simulink model "Main20210122"  (R2021b)
settings: Solver=ode4  StartTime=0.0  StopTime=20  FixedStep=0.0005  RelTol=1e-3  EnableMultiTasking=on
StopFcn:
  | PlotObsError20201214
settings Model: Creator=ysun  LastModifiedBy=yiyon
settings SolverCC: AlgebraicLoopSolver=TrustRegion
settings DataIOCC: LimitDataPoints=on  SaveFormat=Array  ReturnWorkspaceOutputs=off
settings OptimizationCC: LifeSpan=inf
settings DebuggingCC: SFUnexpectedBacktrackingDiag=warning  SFNoUnconditionalDefaultTransitionDiag=warning  SFExecutionAtInitializationDiag=none  SFMachineParentedDataDiag=warning  ArithmeticOperatorsInVariantConditions=warning
settings HardwareCC: ProdBitPerPointer=32  ProdBitPerSizeT=32  ProdBitPerPtrDiffT=32  ProdLargestAtomicFloat=None  ProdIntDivRoundTo=Undefined  ProdEndianess=Unspecified  ProdWordSize=32  ProdHWDeviceType=32-bit Generic
settings ModelReferenceCC: PropagateSignalLabelsOutOfModel=off
settings SFSimCC: SimUseLocalCustomCode=off  CustomCodeUndefinedFunction=UseInterfaceOnly
settings RTWCC: RTWUseLocalCustomCode=off
settings CodeAppCC: StateflowObjectComments=on
settings GRTTargetCC: TargetLangStandard=C89/C90 (ANSI)
settings ConfigComp: CovMetricSettings=dw  CovSaveCumulativeToWorkspaceVar=on  CovSaveSingleToWorkspaceVar=on  CovExternalEMLEnable=off  CovSFcnEnable=off
settings SimscapeCC: SimscapeNormalizeSystem=off
settings ConfigurationSet: Description=SimMechanics 2G

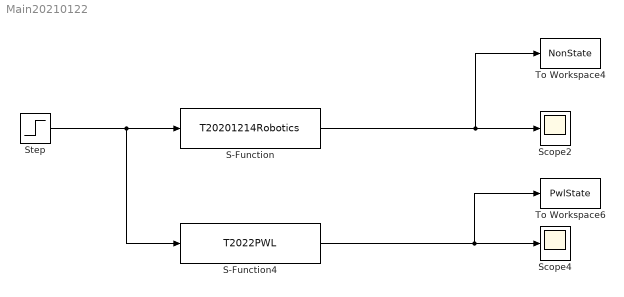
== system Main20210122 ==
  S-Function : S-Function  FunctionName=T20201214Robotics  SFunctionDeploymentMode=off  EnableBusSupport=off
  S-Function4 : S-Function  FunctionName=T2022PWL  SFunctionDeploymentMode=off  EnableBusSupport=off
  Scope2 : Scope
  Scope4 : Scope
  Step : Step  SampleTime=0
  To Workspace4 : ToWorkspace  VariableName=NonState  SaveFormat=Timeseries  SampleTime=-1
  To Workspace6 : ToWorkspace  VariableName=PwlState  SaveFormat=Timeseries  SampleTime=-1
  wires:
  S-Function/1 -> To Workspace4/1, Scope2/1
  Step/1 -> S-Function4/1, S-Function/1
  S-Function4/1 -> To Workspace6/1, Scope4/1
